simulink model "PWM"  (Simulink 7.5)
settings: Solver=FixedStepDiscrete  SolverMode=SingleTasking  StartTime=0.0  StopTime=10.0  FixedStep=0.001  RelTol=1e-3
undefined symbols (not defined in the file or in its folder): Ts
libraries: dsPICdrivers x2, simulink x1
settings Model: Creator=PG Machines Lab  LastModifiedBy=PG Machines Lab
settings OptimizationCC: OptimizeModelRefInitCode=on  LifeSpan=1
settings HardwareCC: ProdBitPerInt=16  ProdEndianess=LittleEndian  ProdWordSize=16  ProdHWDeviceType=16-bit Generic
settings RTWCC: SystemTargetFile=dspic.tlc  TemplateMakefile=dspic_pic30_gcc.tmf  PostCodeGenCommand=dsPIC_Compile()  Description=Embedded Target for Microchip dsPIC (real-time)  ProcessScript=dspic_make_rtw_hook
settings CodeAppCC: IgnoreCustomStorageClasses=off
settings STFCustomTargetCC: IncludeMdlTerminateFcn=off  CombineOutputUpdateFcns=on  SuppressErrorStatus=on  ERTCustomFileBanners=on  SupportContinuousTime=off  SupportNonInlinedSFcns=off  SystemTargetFile=dspic.tlc
settings ERTTargetCC: MultiwordLength=2048  ParMdlRefBuildCompliant=off  CompOptLevelCompliant=off  IncludeMdlTerminateFcn=off  SuppressErrorStatus=on  ERTFirstTimeCompliant=off  ModelStepFunctionPrototypeControlCompliant=off  CPPClassGenCompliant=off  InlinedParameterPlacement=NonHierarchical  ERTSrcFileBannerTemplate=dsPIC_code_template.cgt  ERTHdrFileBannerTemplate=dsPIC_code_template.cgt  ERTDataSrcFileTemplate=dsPIC_code_template.cgt  ERTDataHdrFileTemplate=dsPIC_code_template.cgt  ERTCustomFileTemplate=dsPIC_main.tlc  ConvertIfToSwitch=off
settings CustomProperty: DataType=string  Value=C:\PROGRA~1\MATLAB\R2010a\bin\win32\gmake

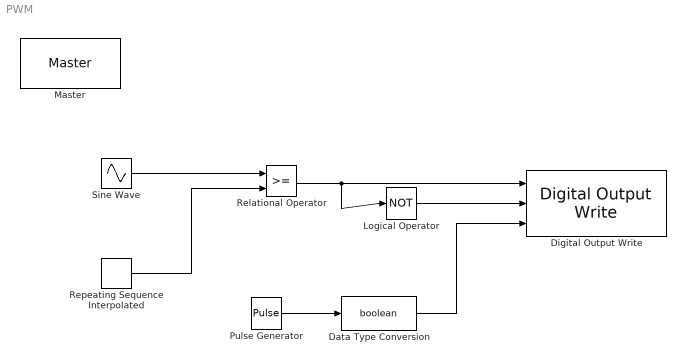
== system PWM ==
  Data Type Conversion : DataTypeConversion  OutDataTypeMode=boolean  OutDataType=fixdt(1, 16)  OutScaling=2^0  OutDataTypeStr=boolean  SampleTime=Ts
  Digital Output Write : dsPICdrivers/Digital I//O/Digital Output Write  Tag=dsPIC_Digital_Output  Priority=5  PORT=D  Pin=[12 14 15]  Simultaneous=off  OrderingInOutPopup=None
  Logical Operator : Logic  Operator=NOT  AllPortsSameDT=off  OutDataTypeMode=boolean  LogicDataType=fixdt(0, 8)  OutDataTypeStr=boolean  SampleTime=Ts
  Master : dsPICdrivers/Master  Tag=dsPIC_MASTER  Priority=1  TimeStepType=Free Run  picType=30f6010  fcy=30e6  Quartz_33f=5e6  PLLActive_33f=off  fcyDesired_33f=0  tmr1="[1  19999  0]"  tmr1Info="Time Step : 0.001  ;   Error : 0%  PR1=29999"  tmr2345="[0  0  0  0]"  tmr2345cfg=[-1 -1 -1 -1]  IOautoConf=on  typePort="[ 0   0   0   0   0   0   0   0   0   0   0   0   0   0   0   0   0   0   0   0   0   0   0   0   0   0   0   0   0   0   0   0   0   0   0   0   0   0   0   0   0   0   0   0   0   0   0   0   0   0   0   0   0   0   0   0   0   0   0   0  10   0  10  10   0   0   0   0   0   0   0   0   0   0   0   0   0   0   0   0   0   0   0   0   0   0   0   0   0   0   0   0   0   0   0   0   0   0   0   0   0   0   0   0   0   0   0   0   0   0   0   0 ]"  TRIS="[ 65535  65535  65535  12287  65535  65535  65535 ]"  ADPCFG=0  MasterBusyPort=None  MasterOverloadPort=None  FOSC=XT_PLL16  ClockSwitchMonitor=Both disabled  TempProtection_33f=TEMP_ON  FPBOR=BORV_20  PWRT=PWRT_OFF  MCLR=MCLR_DIS  ICD=ICS_PGD1  JTAGEN=JTAGEN_OFF  PowerSave=off  OverrideFcy=off  NewFcy=1e6  PR2345="[65535  65535  65535  65535]"
  Pulse Generator : DiscretePulseGenerator  PulseType=Time based  Amplitude=1  Period=Ts  PulseWidth=50  PhaseDelay=0  SampleTime=1
  Relational Operator : RelationalOperator  LogicOutDataTypeMode=boolean  LogicDataType=fixdt(0, 8)  OutDataTypeStr=boolean  SampleTime=Ts
  Repeating Sequence Interpolated : simulink/Sources/Repeating Sequence Interpolated  SystemSampleTime=-1  OutValues=[0 1 -1 0]  TimeValues=[0 5e-5 15e-5 20e-5]  LookUpMeth=Interpolation-Use End Values  tsamp=Ts  OutMin=[]  OutMax=[]  OutDataTypeStr=double  OutputDataTypeScalingMode=double  OutDataType=fixdt(0,8)  OutScaling=2^-10
  Sine Wave : Sin  Amplitude=1  Bias=0  Frequency=2*pi*50  Phase=0  Samples=10  SampleTime=Ts  Offset=0
  wires:
  Sine Wave/1 -> Relational Operator/1
  Repeating Sequence Interpolated/1 -> Relational Operator/2
  Relational Operator/1 -> Digital Output Write/1, Logical Operator/1
  Logical Operator/1 -> Digital Output Write/2
  Pulse Generator/1 -> Data Type Conversion/1
  Data Type Conversion/1 -> Digital Output Write/3
